simulink model "cart_pendulum"  (R2025b)
settings: Solver=ode4  StartTime=0.0  StopTime=p.stopTime  FixedStep=p.sampleTime  RelTol=1e-3
model workspace (MAT data in the model file):
  Ad = [1  0.00199976980145  -3.81082655969e-06  -2.54058914809e-09; 0  0.999769809887  -0.00381072021024  -3.81082655969e-06; 0  6.16608669431e-07  1.00006276169  0.00200004184108; 0  0.000616591461618  0.0627619571552  1.00006276169]
  Bd = [2.87748191952e-06; 0.00287737641237; -7.70760836789e-06; -0.00770739327022]
  C = [1  0  0  0; 0  0  1  0]
  Fkalman = [0.868381113851  0  -3.64301714019e-05  0; -4.37773109331  1  0.00120823606538  0; -0.000198342044299  0  0.896685331295  0; -0.0318825167778  0  -2.7657116556  1]
  I = 0.004704
  Jp = 0.004704
  K = [-13.0634910138 -12.5867192363 -62.5999253657 -11.4912316836]
  M = 0.65
  Mc = 0.65
  Mkalman = [0.131618886149  3.64301714019e-05; 4.37773109331  -0.00120823606538; 0.000198342044299  0.103314668705; 0.0318825167778  2.7657116556]
  Nbar = -13.0634910138
  b = 0.08
  ell = 0.28
  fric = 0.08
  g = 9.81
  grav = 9.81
  l = 0.28
  m = 0.18
  measurementNoise.signals.values = [0.000103093479417 6.74657677723e-06 -5.09485259637e-06 -0.000363482386576 0.000369625102226 -9.79874894757e-05 -0.000369358799553 -0.000421984533503 -0.000205827979281 0.000237630528572 0.000229967262696 -0.000371097329828 ... (5120 elements, 2560x2)]
  measurementNoise.signals.dimensions = 2
  measurementNoise.time = []
  mp = 0.18
  p.cartMass = 0.65
  p.pendulumMass = 0.18
  p.halfLength = 0.28
  p.inertia = 0.004704
  p.cartFriction = 0.08
  p.gravity = 9.81
  p.forceLimit = 8
  p.sampleTime = 0.002
  p.initialState = [0; 0; 0.08; 0]
  p.reference = 0.15
  p.referenceTime = 0.35
  p.disturbanceTime = 3.026
  p.disturbanceDuration = 0.12
  p.disturbanceForce = 0.7
  p.positionNoiseStd = 0.0003
  p.angleNoiseStd = 0.0007
  p.forceNoiseStd = 0.02
  p.seed = 73
  p.stopTime = 5.118
  processForce.signals.values = [-0.0166897120847 0.0305093603326 0.0114415637644 -0.0112851354688 -0.0190319412366 0.0286886342252 0.0129922282298 0.00505032157526 0.00978148544616 -0.0442398361863 0.0293041337753 -0.000945957753953 ... (2560 elements, 2560x1)]
  processForce.signals.dimensions = 1
  processForce.time = []
  useEstimator = 1
values from neighbouring files (symbols this model uses):
  p = project_parameters()    [run_demo.m]
settings Model: Creator=LENOVO  LastModifiedBy=LENOVO

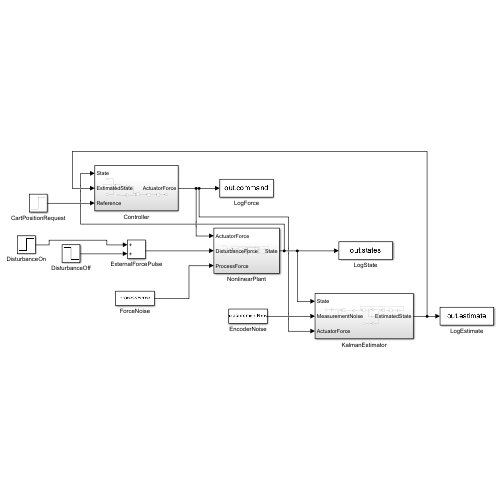
[thumbnail: Simulink's stored preview of the top-level diagram]
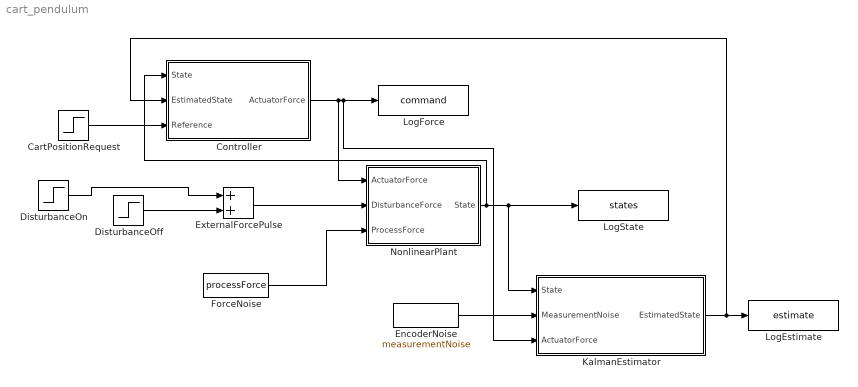
== system cart_pendulum ==
  CartPositionRequest : Step  Time=p.referenceTime  After=p.reference  SampleTime=p.sampleTime
  Controller : Subsystem
  DisturbanceOff : Step  Time=p.disturbanceTime+p.disturbanceDuration  After=-p.disturbanceForce  SampleTime=p.sampleTime
  DisturbanceOn : Step  Time=p.disturbanceTime  After=p.disturbanceForce  SampleTime=p.sampleTime
  EncoderNoise : FromWorkspace  VariableName=measurementNoise  SampleTime=p.sampleTime  Interpolate=off  OutputAfterFinalValue=Holding final value
  ExternalForcePulse : Sum
  ForceNoise : FromWorkspace  VariableName=processForce  SampleTime=p.sampleTime  Interpolate=off  OutputAfterFinalValue=Holding final value
  KalmanEstimator : Subsystem
  LogEstimate : ToWorkspace  VariableName=estimate  SaveFormat=Timeseries  SampleTime=-1
  LogForce : ToWorkspace  VariableName=command  SaveFormat=Timeseries  SampleTime=-1
  LogState : ToWorkspace  VariableName=states  SaveFormat=Timeseries  SampleTime=-1
  NonlinearPlant : Subsystem
  wires:
  Controller/1(ActuatorForce) -> LogForce/1, KalmanEstimator/3(ActuatorForce), NonlinearPlant/1(ActuatorForce)
  KalmanEstimator/1(EstimatedState) -> Controller/2(EstimatedState), LogEstimate/1
  NonlinearPlant/1(State) -> LogState/1, KalmanEstimator/1(State), Controller/1(State)
  EncoderNoise/1 -> KalmanEstimator/2(MeasurementNoise)
  ForceNoise/1 -> NonlinearPlant/3(ProcessForce)
  ExternalForcePulse/1 -> NonlinearPlant/2(DisturbanceForce)
  DisturbanceOff/1 -> ExternalForcePulse/2
  DisturbanceOn/1 -> ExternalForcePulse/1
  CartPositionRequest/1 -> Controller/3(Reference)

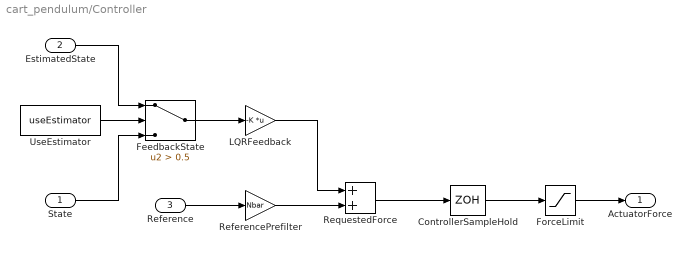
== system cart_pendulum/Controller ==
  State : Inport
  EstimatedState : Inport  Port=2
  Reference : Inport  Port=3
  ControllerSampleHold : ZeroOrderHold  SampleTime=p.sampleTime
  FeedbackState : Switch  Criteria=u2 > Threshold  Threshold=0.5  SaturateOnIntegerOverflow=off  InputSameDT=off
  ForceLimit : Saturate  UpperLimit=p.forceLimit  LowerLimit=-p.forceLimit
  LQRFeedback : Gain  Gain=-K  Multiplication=Matrix(K*u)
  ReferencePrefilter : Gain  Gain=Nbar
  RequestedForce : Sum
  UseEstimator : Constant  Value=useEstimator
  ActuatorForce : Outport
  wires:
  ForceLimit/1 -> ActuatorForce/1
  ControllerSampleHold/1 -> ForceLimit/1
  RequestedForce/1 -> ControllerSampleHold/1
  ReferencePrefilter/1 -> RequestedForce/2
  LQRFeedback/1 -> RequestedForce/1
  Reference/1 -> ReferencePrefilter/1
  FeedbackState/1 -> LQRFeedback/1
  State/1 -> FeedbackState/3
  UseEstimator/1 -> FeedbackState/2
  EstimatedState/1 -> FeedbackState/1

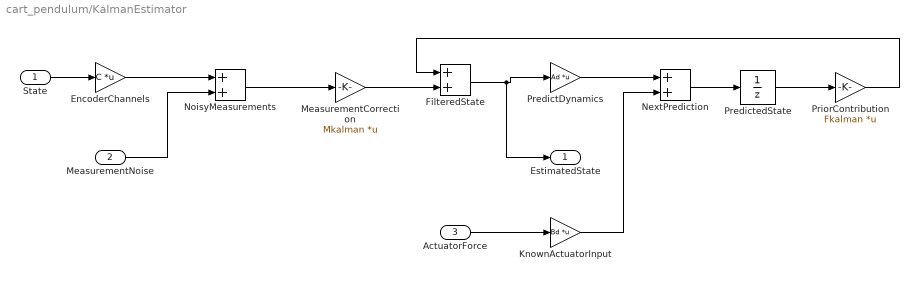
== system cart_pendulum/KalmanEstimator ==
  State : Inport
  MeasurementNoise : Inport  Port=2
  ActuatorForce : Inport  Port=3
  EncoderChannels : Gain  Gain=C  Multiplication=Matrix(K*u)
  FilteredState : Sum
  KnownActuatorInput : Gain  Gain=Bd  Multiplication=Matrix(K*u)
  MeasurementCorrection : Gain  Gain=Mkalman  Multiplication=Matrix(K*u)
  NextPrediction : Sum
  NoisyMeasurements : Sum
  PredictDynamics : Gain  Gain=Ad  Multiplication=Matrix(K*u)
  PredictedState : UnitDelay  InitialCondition=zeros(4,1)  SampleTime=p.sampleTime  HasFrameUpgradeWarning=on
  PriorContribution : Gain  Gain=Fkalman  Multiplication=Matrix(K*u)
  EstimatedState : Outport
  wires:
  NextPrediction/1 -> PredictedState/1
  KnownActuatorInput/1 -> NextPrediction/2
  PredictDynamics/1 -> NextPrediction/1
  ActuatorForce/1 -> KnownActuatorInput/1
  FilteredState/1 -> EstimatedState/1, PredictDynamics/1
  MeasurementCorrection/1 -> FilteredState/2
  PriorContribution/1 -> FilteredState/1
  NoisyMeasurements/1 -> MeasurementCorrection/1
  PredictedState/1 -> PriorContribution/1
  MeasurementNoise/1 -> NoisyMeasurements/2
  EncoderChannels/1 -> NoisyMeasurements/1
  State/1 -> EncoderChannels/1

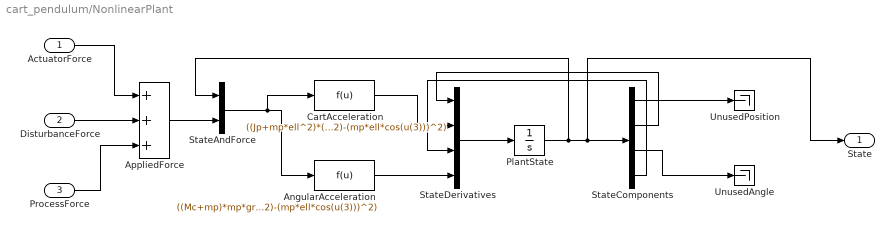
== system cart_pendulum/NonlinearPlant ==
  ActuatorForce : Inport
  DisturbanceForce : Inport  Port=2
  ProcessForce : Inport  Port=3
  AngularAcceleration : Fcn  Expr=((Mc+mp)*mp*grav*ell*sin(u(3))-mp*ell*cos(u(3))*(u(5)-fric*u(2)+mp*ell*u(4)^2*sin(u(3))))/((Mc+mp)*(Jp+mp*ell^2)-(mp*ell*cos(u(3)))^2)
  AppliedForce : Sum  Inputs=+++
  CartAcceleration : Fcn  Expr=((Jp+mp*ell^2)*(u(5)-fric*u(2)+mp*ell*u(4)^2*sin(u(3)))-mp*ell*cos(u(3))*mp*grav*ell*sin(u(3)))/((Mc+mp)*(Jp+mp*ell^2)-(mp*ell*cos(u(3)))^2)
  PlantState : Integrator  InitialCondition=p.initialState
  StateAndForce : Mux  Inputs=2
  StateComponents : Demux
  StateDerivatives : Mux
  UnusedAngle : Terminator
  UnusedPosition : Terminator
  State : Outport
  wires:
  StateComponents/3 -> UnusedAngle/1
  StateComponents/1 -> UnusedPosition/1
  StateDerivatives/1 -> PlantState/1
  AngularAcceleration/1 -> StateDerivatives/4
  StateComponents/4 -> StateDerivatives/3
  CartAcceleration/1 -> StateDerivatives/2
  StateComponents/2 -> StateDerivatives/1
  StateAndForce/1 -> CartAcceleration/1, AngularAcceleration/1
  AppliedForce/1 -> StateAndForce/2
  PlantState/1 -> StateComponents/1, State/1, StateAndForce/1
  ProcessForce/1 -> AppliedForce/3
  DisturbanceForce/1 -> AppliedForce/2
  ActuatorForce/1 -> AppliedForce/1
